simulink subsystem "ctrl_hybrid"  (R2026a)
settings: Solver=VariableStepAuto
undefined symbols (not defined in the file or in its folder): ctrlP, hcfg
libraries: simulink x1
settings Model: Creator=ahmad  LastModifiedBy=ahmad

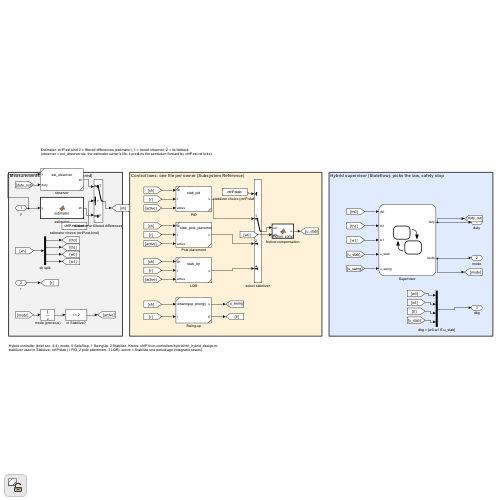
[thumbnail: Simulink's stored preview of the top-level diagram]
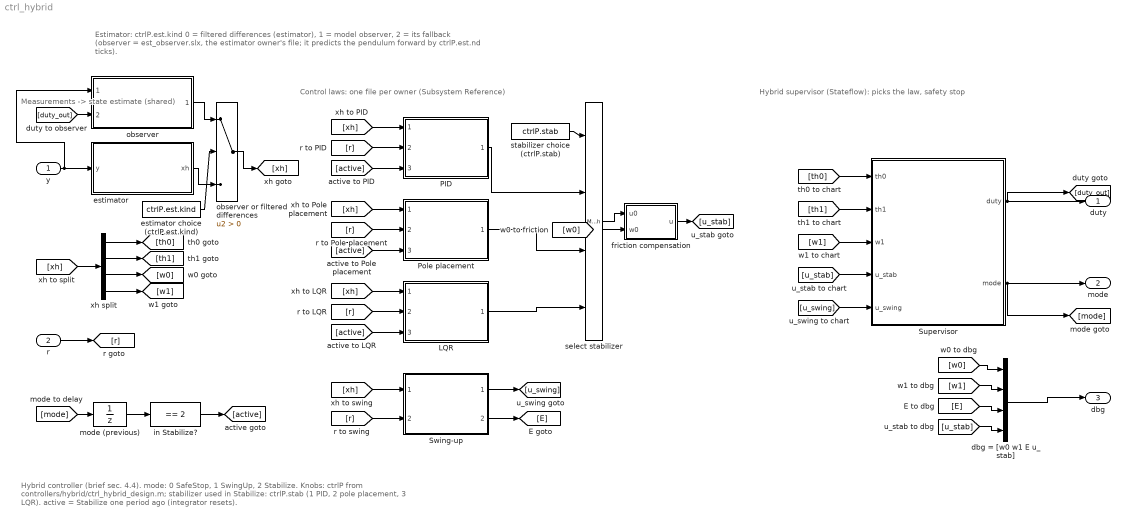
== system ctrl_hybrid ==
  note: Measurements -> state estimate (shared)
  note: Control laws: one file per owner (Subsystem Reference)
  note: Hybrid supervisor (Stateflow): picks the law, safety stop
  note: Hybrid controller (brief sec. 4.4). mode: 0 SafeStop, 1 SwingUp, 2 Stabilize. Knobs: ctrlP from controllers/hybrid/ctrl_hybrid_design.m;
      | stabilizer used in Stabilize: ctrlP.stab (1 PID, 2 pole placement, 3 LQR). active = Stabilize one period ago (integrator resets).
  note: Estimator: ctrlP.est.kind 0 = filtered differences (estimator), 1 = model observer, 2 = its fallback
      | (observer = est_observer.slx, the estimator owner's file; it predicts the pendulum forward by ctrlP.est.nd ticks).
  y : Inport  PortDimensions=3  SampleTime=hcfg.Ts
  r : Inport  Port=2
  LQR : Subsystem  ReferencedSubsystem=stab_lqr
  PID : Subsystem  ReferencedSubsystem=stab_pid
  Pole placement : Subsystem  ReferencedSubsystem=stab_pole_placement
  Supervisor : Stateflow chart  TreatAsAtomicUnit=on
  Swing-up : Subsystem  ReferencedSubsystem=swingup_energy
  dbg = [w0 w1 E u_stab] : Mux
  estimator : MATLAB Function  TreatAsAtomicUnit=on
  estimator choice (ctrlP.est.kind) : Constant  Value=ctrlP.est.kind
  friction compensation : MATLAB Function  TreatAsAtomicUnit=on
  in Stabilize? : simulink/Logic and Bit Operations/Compare To Constant  relop===  const=2  OutDataTypeStr=boolean
  mode (previous) : UnitDelay  SampleTime=hcfg.Ts
  observer : Subsystem  ReferencedSubsystem=est_observer
  observer or filtered differences : Switch  Criteria=u2 > Threshold  SaturateOnIntegerOverflow=off  InputSameDT=off
  select stabilizer : MultiPortSwitch  SaturateOnIntegerOverflow=off  InputSameDT=off
  stabilizer choice (ctrlP.stab) : Constant  Value=ctrlP.stab
  xh split : Demux
  duty : Outport
  mode : Outport  Port=2
  dbg : Outport  Port=3
  wires:
  y/1 -> estimator/1(y), observer/1
  [xh] -> xh split/1
  xh split/1 -> [th0]
  xh split/2 -> [th1]
  xh split/3 -> [w0]
  xh split/4 -> [w1]
  r/1 -> [r]
  [mode] -> mode (previous)/1
  mode (previous)/1 -> in Stabilize?/1
  in Stabilize?/1 -> [active]
  [xh] -> PID/1
  [r] -> PID/2
  [active] -> PID/3
  [xh] -> Pole placement/1
  [r] -> Pole placement/2
  [active] -> Pole placement/3
  [xh] -> LQR/1
  [r] -> LQR/2
  [active] -> LQR/3
  [xh] -> Swing-up/1
  [r] -> Swing-up/2
  Swing-up/1 -> [u_swing]
  Swing-up/2 -> [E]
  stabilizer choice (ctrlP.stab)/1 -> select stabilizer/1
  PID/1 -> select stabilizer/2
  Pole placement/1 -> select stabilizer/3
  LQR/1 -> select stabilizer/4
  select stabilizer/1 -> friction compensation/1(u0)
  friction compensation/1(u) -> [u_stab]
  [th0] -> Supervisor/1(th0)
  [th1] -> Supervisor/2(th1)
  [w1] -> Supervisor/3(w1)
  [u_stab] -> Supervisor/4(u_stab)
  [u_swing] -> Supervisor/5(u_swing)
  Supervisor/1(duty) -> duty/1, [duty_out]
  Supervisor/2(mode) -> mode/1, [mode]
  [w0] -> dbg = [w0 w1 E u_stab]/1
  [w1] -> dbg = [w0 w1 E u_stab]/2
  [E] -> dbg = [w0 w1 E u_stab]/3
  [u_stab] -> dbg = [w0 w1 E u_stab]/4
  dbg = [w0 w1 E u_stab]/1 -> dbg/1
  [w0] -> friction compensation/2(w0)
  [duty_out] -> observer/2
  observer/1 -> observer or filtered differences/1
  estimator choice (ctrlP.est.kind)/1 -> observer or filtered differences/2
  estimator/1(xh) -> observer or filtered differences/3
  observer or filtered differences/1 -> [xh]

== matlab function ctrl_hybrid/estimator ==
  data: y input; xh output; ctrlP parameter
function xh = estimator(y, ctrlP)
% xh = [theta0; theta1 wrapped to [-pi, pi) (0 = up); dtheta0; dtheta1]
% Velocities: finite differences low-pass filtered at ctrlP.est.vel_fc. Replace with an
% observer (e.g. Kalman) if you like; keep the output.
persistent prev w
th = [y(1); mod(y(2) + pi, 2*pi) - pi];
if isempty(prev)
    prev = th; w = [0; 0];
end
a = exp(-2*pi*ctrlP.est.vel_fc*ctrlP.Ts);
d = th - prev;
d(2) = mod(d(2) + pi, 2*pi) - pi;                % no jump when theta1 wraps
w = a*w + (1 - a)*d/ctrlP.Ts;
prev = th;
xh = [th; w];

== matlab function ctrl_hybrid/friction compensation ==
  data: u0 input; w0 input; u output; ctrlP parameter
function u = friction_comp(u0, w0, ctrlP)
% Friction compensation on the stabilizer output, in the direction of the request (smooth sign of u0):
% the identified Coulomb duty (report 5.7) while the arm slides, blending to the breakaway duty
% (13 % / 14 %, measured) when the arm is at rest (firmware 1.9). With Coulomb only, the LQR's small
% corrections stuck below the breakaway on the rig (run 20261119_205453). fric.gain 0 = off,
% fric.stick 0 = Coulomb only. The fade width is the swing-up's w_stick, as in the firmware.
s = tanh(u0/ctrlP.fric.band);
coul = ctrlP.fric.duty(1)*max(s, 0) + ctrlP.fric.duty(2)*min(s, 0);
stat = ctrlP.fric.stick_duty(1)*max(s, 0) + ctrlP.fric.stick_duty(2)*min(s, 0);
g = exp(-(w0/ctrlP.swing.w_stick)^2);
u = u0 + ctrlP.fric.gain*(coul + ctrlP.fric.stick*g*(stat - coul));

== stateflow chart ctrl_hybrid/Supervisor ==
  state SwingUp
    en, du:
    mode = 1;
    duty = u_swing;
  state Stabilize
    en, du:
    mode = 2;
    duty = u_stab;
  state SafeStop
    en, du:
    mode = 0;
    duty = 0;
  (default) -> (junction 12)
  (junction 12) -> SwingUp [order 2]
  (junction 12) -> Stabilize [order 1] : [abs(th1) < ctrlP.sup.catch_th1 && abs(w1) < ctrlP.sup.catch_w1]
  SwingUp -> Stabilize [order 2] : [abs(th1) < ctrlP.sup.catch_th1 && abs(w1) < ctrlP.sup.catch_w1]
  Stabilize -> SwingUp [order 2] : [abs(th1) > ctrlP.sup.exit_th1]
  SafeStop -> SwingUp : [ctrlP.sup.rearm && abs(th0) < ctrlP.sup.safe_th0/2 && abs(th1) > pi - 0.2 && abs(w1) < 0.5]
  SwingUp -> SafeStop [order 1] : [abs(th0) > ctrlP.sup.safe_th0]
  Stabilize -> SafeStop [order 1] : [abs(th0) > ctrlP.sup.safe_th0]
  data: th0 input; th1 input; w1 input; u_stab input; u_swing input; duty output double; mode output double; ctrlP parameter
